simulink model "Practica4_MSF1_MAT"  (R2024b)
settings: Solver=VariableStepAuto  StartTime=0.0  StopTime=10.0  RelTol=1e-3
libraries: slpidlib x1
settings Model: Creator=ASUS  LastModifiedBy=Angel Torales
settings DataIOCC: SaveOutput=off  SignalLogging=off  DSMLogging=off  ReturnWorkspaceOutputs=off  TimeSaveName=t
settings DebuggingCC: AlgebraicLoopMsg=none  ArtificialAlgebraicLoopMsg=none  MaxConsecutiveZCsMsg=none  OperatingPointInterfaceChecksumMismatchMsg=none

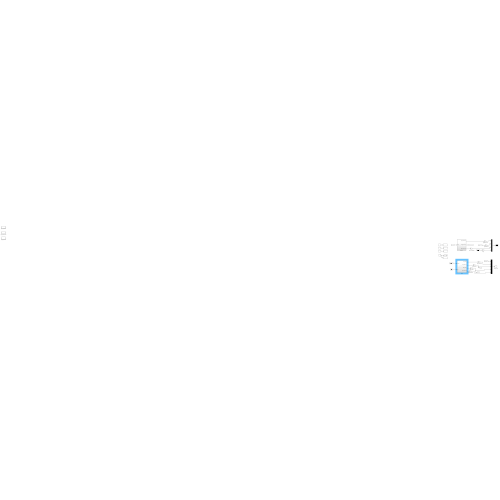
[thumbnail: Simulink's stored preview of the top-level diagram]
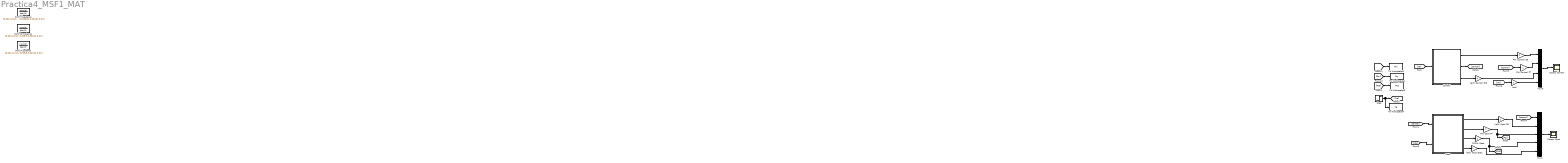
== system Practica4_MSF1_MAT ==
  " Pp(t):Hipertenso" : TransferFcn  Numerator=[0.001,0.01]  Denominator=[0.00001,0.00101,0.01]
  " Pp(t):Hipotenso" : TransferFcn  Numerator=[0.001,0.01]  Denominator=[3.5E-5,0.00101,0.01]
  " Pp(t):Normotenso" : TransferFcn  Numerator=[0.001,0.01]  Denominator=[1.5E-5,0.00101,0.01]
  Caso : Subsystem
  Control : Subsystem
  F(t): Caso FT : Gain
  F(t): Control CE : Gain
  F(t): Control FT : Gain
  Mux2 : Mux  Inputs=5
  Mux3 : Mux
  PID(t): Caso : Gain
  Scope: Caso : Scope
  Scope: Control : Scope
  Step : Step  Time=0  SampleTime=0
  To Workspace1 : ToWorkspace  VariableName=Fsx  SampleTime=-1
  To Workspace2 : ToWorkspace  VariableName=Fsy  SampleTime=-1
  To Workspace3 : ToWorkspace  VariableName=PID  SampleTime=-1
  To Workspace4 : ToWorkspace  VariableName=Ve  SampleTime=-1
  Ve(t) : Gain
  Ve(t): Caso CE : Gain
  Ve(t): Caso EID1 : Gain
  Ve(t): Control EID : Gain
  wires:
  [Ve] -> Control/1(Ve(t))
  Mux2/1 -> Scope: Caso/1
  F(t): Caso FT/1 -> [Fsy], Mux2/3
  Mux3/1 -> Scope: Control/1
  [control] -> F(t): Control FT/1
  [control] -> To Workspace1/1
  [Fsy] -> To Workspace2/1
  Control/2(Ve(t): Control FT) -> [control]
  [control] -> Caso/1(Control)
  Caso/2(Ve(t): Caso FT) -> F(t): Caso FT/1
  [control] -> Mux2/1
  PID(t): Caso/1 -> [PID], Mux2/4
  Caso/3(PID(t): Caso) -> PID(t): Caso/1
  [PID] -> To Workspace3/1
  [Ve] -> Caso/2(F(t))
  Ve(t): Caso CE/1 -> Mux2/2
  Caso/1(Vs(t): Caso) -> Ve(t): Caso CE/1
  F(t): Control FT/1 -> Mux3/2
  F(t): Control CE/1 -> Mux3/1
  Control/1(Ve(t): Control CE) -> F(t): Control CE/1
  Step/1 -> To Workspace4/1, [Ve]
  Ve(t): Control EID/1 -> Mux3/3
  Control/3(Ve(t): Control EID) -> Ve(t): Control EID/1
  Caso/4(Ve(t): Caso EID) -> Ve(t): Caso EID1/1
  Ve(t): Caso EID1/1 -> Mux2/5
  Ve(t)/1 -> Mux3/4
  [Ve] -> Ve(t)/1

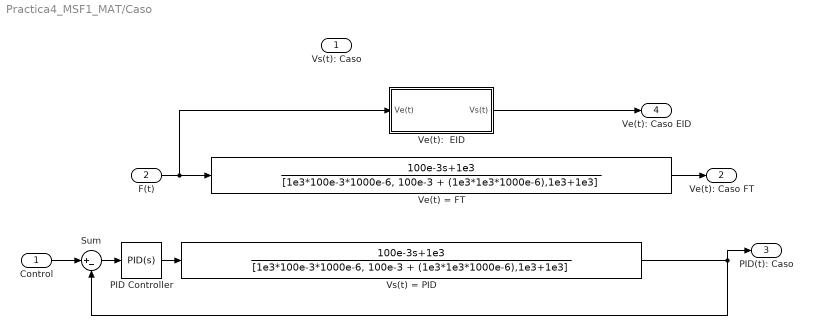
== system Practica4_MSF1_MAT/Caso ==
  Control : Inport
  F(t) : Inport  Port=2
  " Ve(t) = FT" : TransferFcn  Numerator=[100e-3,1e3]  Denominator=[1e3*100e-3*1000e-6, 100e-3 + (1e3*1e3*1000e-6),1e3+1e3]
  " Vs(t) = PID" : TransferFcn  Numerator=[100e-3,1e3]  Denominator=[1e3*100e-3*1000e-6, 100e-3 + (1e3*1e3*1000e-6),1e3+1e3]
  PID Controller : slpidlib/PID Controller  Controller=PID  Form=Parallel  TimeDomain=Continuous-time  UseExternalTs=off  SampleTime=-1  IntegratorMethod=Forward Euler  FilterMethod=Forward Euler  ControllerParametersSource=internal  P=19075.4868097833  I=67385555.4118663  UseKiTs=off  D=0.181174004730977  UseExternalDerivativeSource=off  N=72936.4813354201  UseFilter=on  TunerSelectOption=Transfer Function Based (PID Tuner App)  InitialConditionSource=internal  InitialConditionForIntegrator=0  InitialConditionForFilter=0  DifferentiatorICPrevScaledInput=0  ExternalReset=none  TrackingMode=off  Kt=1  LimitOutput=off  SatLimitsSource=internal  UpperSaturationLimit=inf  LowerSaturationLimit=-inf  LinearizeAsGain=on  AntiWindupMode=none  Kb=1  LimitIntegrator=off  UpperIntegratorSaturationLimit=inf  LowerIntegratorSaturationLimit=-inf  POutMin=[]  POutMax=[]  IOutMin=[]  IOutMax=[]  DOutMin=[]  DOutMax=[]  NOutMin=[]  NOutMax=[]  SumOutMin=[]  SumOutMax=[]  SaturationOutMin=[]  SaturationOutMax=[]  PParamMin=[]  PParamMax=[]  IParamMin=[]  IParamMax=[]  DParamMin=[]  DParamMax=[]  NParamMin=[]  NParamMax=[]  KbParamMin=[]  KbParamMax=[]  KtParamMin=[]  KtParamMax=[]  KbOutMin=[]  KbOutMax=[]  KtOutMin=[]  KtOutMax=[]  IntegratorOutMin=[]  IntegratorOutMax=[]  FilterOutMin=[]  FilterOutMax=[]  SumI1OutMin=[]  SumI1OutMax=[]  SumI2OutMin=[]  SumI2OutMax=[]  SumI3OutMin=[]  SumI3OutMax=[]  SumI4OutMin=[]  SumI4OutMax=[]  SumDOutMin=[]  SumDOutMax=[]  DifferentiatorOutMin=[]  DifferentiatorOutMax=[]  FilterDiffOutCoefMin=[]  FilterDiffOutCoefMax=[]  ReciprocalOutMin=[]  ReciprocalOutMax=[]  SumDenOutMin=[]  SumDenOutMax=[]  SumNumOutMin=[]  SumNumOutMax=[]  DivideOutMin=[]  DivideOutMax=[]  UdiffTsProdOutMin=[]  UdiffTsProdOutMax=[]  NTsProdOutMin=[]  NTsProdOutMax=[]  UintegralTsProdOutMin=[]  UintegralTsProdOutMax=[]  UngainTsProdOutMin=[]  UngainTsProdOutMax=[]  ClampingZeroOutDataTypeStr=Inherit: Inherit via back propagation  ClampingZeroOutMin=[]  ClampingZeroOutMax=[]  FilterDenConstantOutDataTypeStr=Inherit: Inherit via back propagation  FilterDenConstantOutMin=[]  FilterDenConstantOutMax=[]  PCopyOutDataTypeStr=Inherit: Inherit via back propagation  PCopyOutMin=[]  PCopyOutMax=[]  NCopyOutDataTypeStr=Inherit: Inherit via back propagation  NCopyOutMin=[]  NCopyOutMax=[]  IntegratorContinuousStateAttributes=''  IntegratorStateMustResolveToSignalObject=off  IntegratorRTWStateStorageClass=Auto  FilterContinuousStateAttributes=''  FilterStateMustResolveToSignalObject=off  FilterRTWStateStorageClass=Auto  ParallelPVariant=InternalParameters  IdealPVariant=Disabled  IVariant=InternalParameters  DVariant=InternalParameters  IntegratorVariant=Continuous  SatVariant=Disabled  AWVariant=Passthrough  PCopyVariant=Disabled  TRVariant=Disabled  FdbkBlocksVariant=Forward  IdealPFdbkVariant=Disabled  SatFdbkVariant=Disabled  DerivativeFilterVariant=ContFilter  NVariant=InternalParameters  NCopyVariant=Disabled  FilterICVariant=InternalICsFilter  IntegratorICVariant=InternalICs  ExternalResetVariant=Disabled  TRSumVariant=Passthrough  SumFdbkVariant=Disabled  SumVariant=Sum_PID  TsampFilterVariant=InternalTs  TsampNgainVariant=Passthrough  TsampIntegralVariant=Disabled_SignalSpec  ExternalSaturationOutDataTypeStr=Inherit: Same as second input  DerivativeSourceVariant=ErrorSignal  PreIntVariant=InternalPreInt
  Sum : Sum  Inputs=|+-
  Ve(t):  EID : Subsystem
  Vs(t): Caso : Outport
  Ve(t): Caso FT : Outport  Port=2
  PID(t): Caso : Outport  Port=3
  Ve(t): Caso EID : Outport  Port=4
  wires:
  " Vs(t) = PID"/1 -> Sum/2, PID(t): Caso/1
  PID Controller/1 -> " Vs(t) = PID"/1
  Sum/1 -> PID Controller/1
  Control/1 -> Sum/1
  F(t)/1 -> Ve(t):  EID/1(Ve(t)), " Ve(t) = FT"/1
  " Ve(t) = FT"/1 -> Ve(t): Caso FT/1
  Ve(t):  EID/1(Vs(t)) -> Ve(t): Caso EID/1

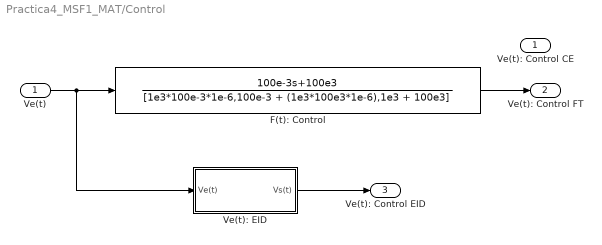
== system Practica4_MSF1_MAT/Control ==
  Ve(t) : Inport
  " F(t): Control" : TransferFcn  Numerator=[100e-3,100e3]  Denominator=[1e3*100e-3*1e-6,100e-3 + (1e3*100e3*1e-6),1e3 + 100e3]
  Ve(t): EID : Subsystem
  Ve(t): Control CE : Outport
  Ve(t): Control FT : Outport  Port=2
  Ve(t): Control EID : Outport  Port=3
  wires:
  Ve(t)/1 -> Ve(t): EID/1(Ve(t)), " F(t): Control"/1
  " F(t): Control"/1 -> Ve(t): Control FT/1
  Ve(t): EID/1(Vs(t)) -> Ve(t): Control EID/1

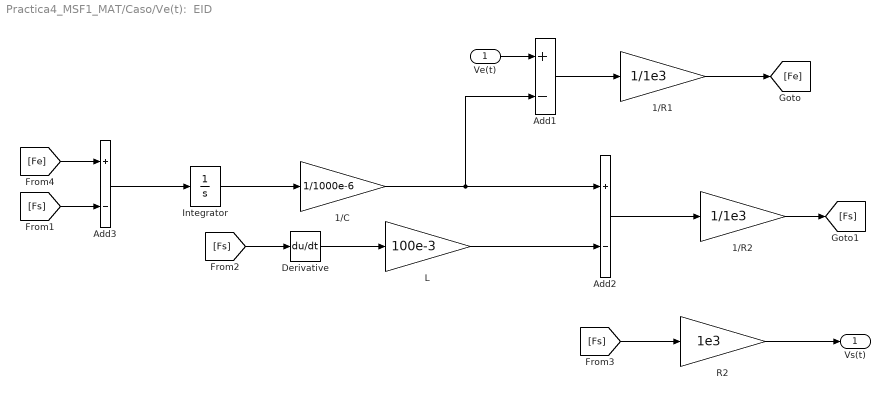
== system Practica4_MSF1_MAT/Caso/Ve(t):  EID ==
  Ve(t) : Inport
  1/C : Gain  Gain=1/1000e-6
  1/R1 : Gain  Gain=1/1e3
  1/R2 : Gain  Gain=1/1e3
  Add1 : Sum  Inputs=+-
  Add2 : Sum  Inputs=+-
  Add3 : Sum  Inputs=+-
  Derivative : Derivative
  Integrator : Integrator
  L : Gain  Gain=100e-3
  R2 : Gain  Gain=1e3
  Vs(t) : Outport
  wires:
  [Fe] -> Add3/1
  [Fs] -> Add3/2
  Ve(t)/1 -> Add1/1
  Add3/1 -> Integrator/1
  Integrator/1 -> 1/C/1
  1/C/1 -> Add1/2, Add2/1
  Derivative/1 -> L/1
  [Fs] -> Derivative/1
  L/1 -> Add2/2
  [Fs] -> R2/1
  Add1/1 -> 1/R1/1
  1/R1/1 -> [Fe]
  Add2/1 -> 1/R2/1
  R2/1 -> Vs(t)/1
  1/R2/1 -> [Fs]

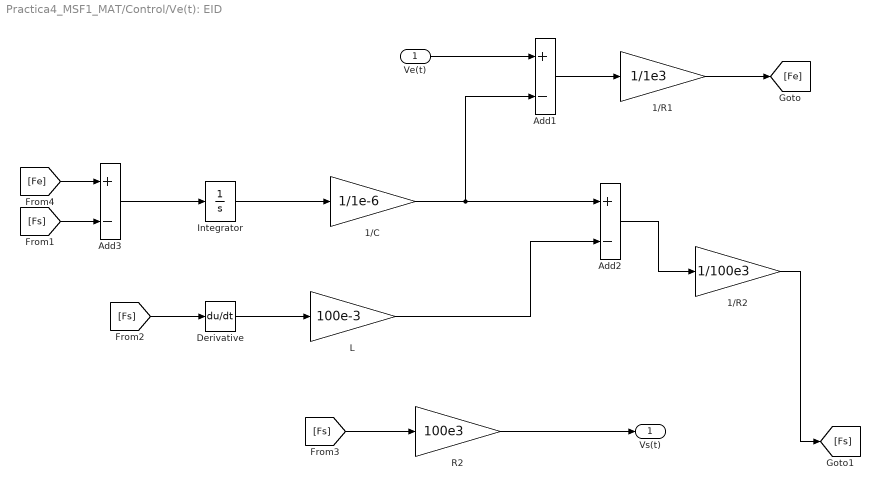
== system Practica4_MSF1_MAT/Control/Ve(t): EID ==
  Ve(t) : Inport
  1/C : Gain  Gain=1/1e-6
  1/R1 : Gain  Gain=1/1e3
  1/R2 : Gain  Gain=1/100e3
  Add1 : Sum  Inputs=+-
  Add2 : Sum  Inputs=+-
  Add3 : Sum  Inputs=+-
  Derivative : Derivative
  Integrator : Integrator
  L : Gain  Gain=100e-3
  R2 : Gain  Gain=100e3
  Vs(t) : Outport
  wires:
  [Fe] -> Add3/1
  [Fs] -> Add3/2
  Ve(t)/1 -> Add1/1
  Add3/1 -> Integrator/1
  Integrator/1 -> 1/C/1
  1/C/1 -> Add1/2, Add2/1
  Derivative/1 -> L/1
  [Fs] -> Derivative/1
  L/1 -> Add2/2
  [Fs] -> R2/1
  Add1/1 -> 1/R1/1
  1/R1/1 -> [Fe]
  Add2/1 -> 1/R2/1
  R2/1 -> Vs(t)/1
  1/R2/1 -> [Fs]
